simulink model "UAV_Hover_Sim"  (R2025b)
settings: Solver=VariableStepAuto  StartTime=0.0  StopTime=inf  RelTol=1e-3
undefined symbols (not defined in the file): A, b0, g, h, quad_m, rho_water, W, wc, wo
libraries: slpidlib x1, aerolibanimutils x1, uavutilslib x1
settings Model: Creator=Aorus PC  LastModifiedBy=David
settings OptimizationCC: ReuseModelBlockBuffer=off
settings DebuggingCC: UnderspecifiedInitializationDetection=Classic  MergeDetectMultiDrivingBlocksExec=none
settings ModelReferenceCC: PropagateSignalLabelsOutOfModel=off
settings RTWCC: GPUComputeCapability=3.5

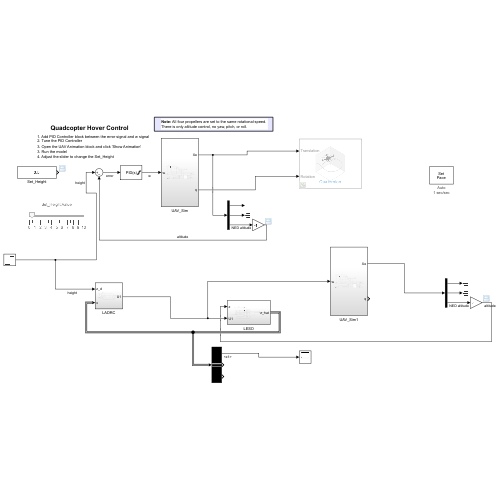
[thumbnail: Simulink's stored preview of the top-level diagram]
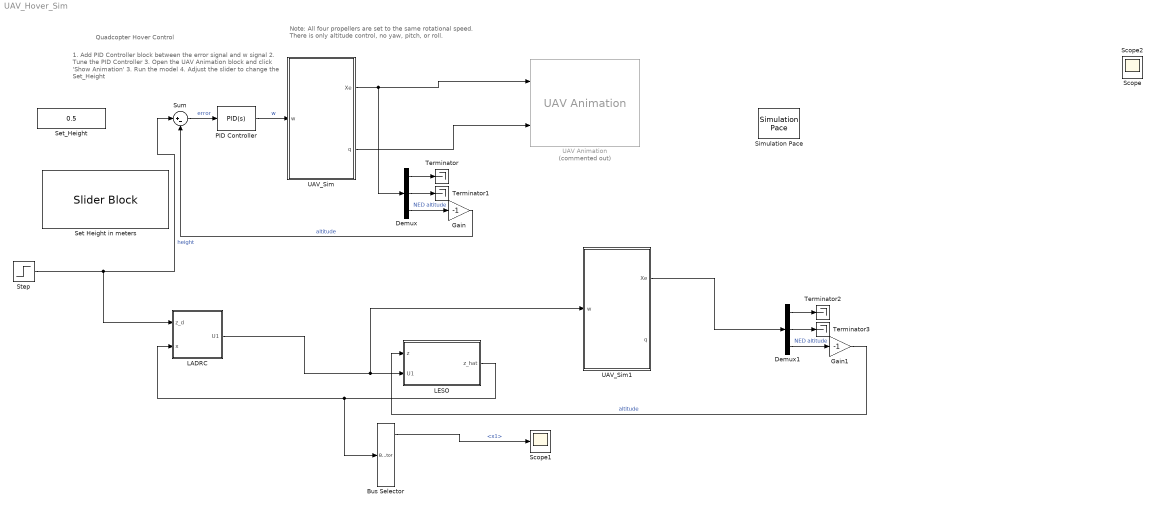
== system UAV_Hover_Sim ==
  note: Note: All four propellers are set to the same rotational speed.
      | There is only altitude control, no yaw, pitch, or roll.
  note: 1. Add PID Controller block between the error signal and w signal 2. Tune the PID Controller
      | 3. Open the UAV Animation block and click 'Show Animation'
      | 3. Run the model
      | 4. Adjust the slider to change the Set_Height
  note: Quadcopter Hover Control
  Bus Selector : BusSelector  OutputSignals=x1,x2,x3
  Demux : Demux  Outputs=3
  Demux1 : Demux  Outputs=3
  Gain : Gain  Gain=-1
  Gain1 : Gain  Gain=-1
  LADRC : Subsystem
  LESO : Subsystem
  PID Controller : slpidlib/PID Controller  Controller=PID  Form=Parallel  TimeDomain=Continuous-time  UseExternalTs=off  SampleTime=-1  IntegratorMethod=Forward Euler  FilterMethod=Forward Euler  ControllerParametersSource=internal  P=20  I=1  UseKiTs=off  D=40  UseExternalDerivativeSource=off  N=10  UseFilter=on  TunerSelectOption=Transfer Function Based (PID Tuner App)  InitialConditionSource=internal  InitialConditionForIntegrator=4000  InitialConditionForFilter=0  DifferentiatorICPrevScaledInput=0  ExternalReset=none  TrackingMode=off  Kt=1  LimitOutput=on  SatLimitsSource=internal  UpperSaturationLimit=10000  LowerSaturationLimit=0  LinearizeAsGain=on  AntiWindupMode=back-calculation  Kb=1  LimitIntegrator=on  UpperIntegratorSaturationLimit=10000  LowerIntegratorSaturationLimit=0  POutMin=[]  POutMax=[]  IOutMin=[]  IOutMax=[]  DOutMin=[]  DOutMax=[]  NOutMin=[]  NOutMax=[]  SumOutMin=[]  SumOutMax=[]  SaturationOutMin=[]  SaturationOutMax=[]  PParamMin=[]  PParamMax=[]  IParamMin=[]  IParamMax=[]  DParamMin=[]  DParamMax=[]  NParamMin=[]  NParamMax=[]  KbParamMin=[]  KbParamMax=[]  KtParamMin=[]  KtParamMax=[]  KbOutMin=[]  KbOutMax=[]  KtOutMin=[]  KtOutMax=[]  IntegratorOutMin=[]  IntegratorOutMax=[]  FilterOutMin=[]  FilterOutMax=[]  SumI1OutMin=[]  SumI1OutMax=[]  SumI2OutMin=[]  SumI2OutMax=[]  SumI3OutMin=[]  SumI3OutMax=[]  SumI4OutMin=[]  SumI4OutMax=[]  SumDOutMin=[]  SumDOutMax=[]  DifferentiatorOutMin=[]  DifferentiatorOutMax=[]  FilterDiffOutCoefMin=[]  FilterDiffOutCoefMax=[]  ReciprocalOutMin=[]  ReciprocalOutMax=[]  SumDenOutMin=[]  SumDenOutMax=[]  SumNumOutMin=[]  SumNumOutMax=[]  DivideOutMin=[]  DivideOutMax=[]  UdiffTsProdOutMin=[]  UdiffTsProdOutMax=[]  NTsProdOutMin=[]  NTsProdOutMax=[]  UintegralTsProdOutMin=[]  UintegralTsProdOutMax=[]  UngainTsProdOutMin=[]  UngainTsProdOutMax=[]  ClampingZeroOutDataTypeStr=Inherit: Inherit via back propagation  ClampingZeroOutMin=[]  ClampingZeroOutMax=[]  FilterDenConstantOutDataTypeStr=Inherit: Inherit via back propagation  FilterDenConstantOutMin=[]  FilterDenConstantOutMax=[]  PCopyOutDataTypeStr=Inherit: Inherit via back propagation  PCopyOutMin=[]  PCopyOutMax=[]  NCopyOutDataTypeStr=Inherit: Inherit via back propagation  NCopyOutMin=[]  NCopyOutMax=[]  IntegratorContinuousStateAttributes=''  IntegratorStateMustResolveToSignalObject=off  IntegratorRTWStateStorageClass=Auto  FilterContinuousStateAttributes=''  FilterStateMustResolveToSignalObject=off  FilterRTWStateStorageClass=Auto  ParallelPVariant=InternalParameters  IdealPVariant=Disabled  IVariant=InternalParameters  DVariant=InternalParameters  IntegratorVariant=Continuous  SatVariant=Enabled  AWVariant=BackCalculation  PCopyVariant=Disabled  TRVariant=Disabled  FdbkBlocksVariant=Forward  IdealPFdbkVariant=Disabled  SatFdbkVariant=Disabled  DerivativeFilterVariant=ContFilter  NVariant=InternalParameters  NCopyVariant=Disabled  FilterICVariant=InternalICsFilter  IntegratorICVariant=InternalICs  ExternalResetVariant=Disabled  TRSumVariant=Passthrough  SumFdbkVariant=Disabled  SumVariant=Sum_PID  TsampFilterVariant=InternalTs  TsampNgainVariant=Passthrough  TsampIntegralVariant=Disabled_SignalSpec  ExternalSaturationOutDataTypeStr=Inherit: Same as second input  DerivativeSourceVariant=ErrorSignal  PreIntVariant=InternalPreInt
  Scope1 : Scope
      settings: ActiveDisplayYMinimum=-1  ActiveDisplayYMaximum=1  DataLoggingVariableName=ScopeData3
  Set Height in meters : SliderBlock  ScaleMax=10  TickInterval=1
  Set_Height : Constant  Value=0.5
  Simulation Pace : aerolibanimutils/Simulation Pace  SimulationPace=1  SleepMode=Auto  OutputPaceError=off  SampleTime=1/30
  Step : Step  Time=10  Before=0.1  After=0.5  SampleTime=0
  Sum : Sum  Inputs=|+-
  Terminator{,1..3} (4 alike) : Terminator
  UAV Animation : uavutilslib/UAV Animation  Commented=on  NumUAV=1  DynamicUAVConfig=off  UAVType=Multirotor  UAVSize=4  UAVColor=[1 0 0]  UAVTrajectoryAlpha=1  InertialZDirection=Down  RotationFormat=Quaternion  DrawMarkers=off  SampleTime=-1
  UAV_Sim : Subsystem
  UAV_Sim1 : Subsystem
  Scope : Scope
      settings: TimeSpan=20  ActiveDisplayYMinimum=0.050000000000000017  ActiveDisplayYMaximum=0.55  YLabel=Altitude (m)
  Scope2 : Scope
      settings: ActiveDisplayYMinimum=0.03970156153398724  ActiveDisplayYMaximum=0.69900672000541475
  wires:
  UAV_Sim/1(Xe) -> Demux/1, UAV Animation/1
  UAV_Sim/2(q) -> UAV Animation/2
  Demux/1 -> Terminator/1
  Demux/2 -> Terminator1/1
  Gain/1 -> Sum/2  "altitude"
  Step/1 -> Sum/1, LADRC/1(z_d)  "height"
  Demux/3 -> Gain/1  "NED altitude"
  PID Controller/1 -> UAV_Sim/1(w)  "w"
  Sum/1 -> PID Controller/1  "error"
  LESO/1(z_hat) -> Bus Selector/1, LADRC/2(x)
  LADRC/1(U1) -> UAV_Sim1/1(w), LESO/2(U1)
  Demux1/3 -> Gain1/1  "NED altitude"
  Demux1/2 -> Terminator3/1
  Demux1/1 -> Terminator2/1
  UAV_Sim1/1(Xe) -> Demux1/1
  Gain1/1 -> LESO/1(z)  "altitude"
  Bus Selector/1 -> Scope1/1  "<x1>"

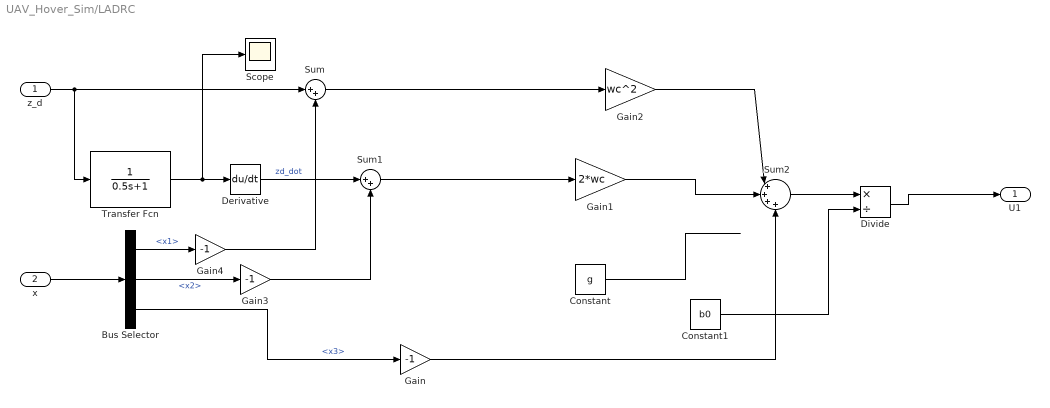
== system UAV_Hover_Sim/LADRC ==
  z_d : Inport
  x : Inport  Port=2
  Bus Selector : BusSelector  OutputSignals=x1,x2,x3
  Constant : Constant  Value=g
  Constant1 : Constant  Value=b0
  Derivative : Derivative
  Divide : Product  Inputs=*/
  Gain : Gain  Gain=-1
  Gain1 : Gain  Gain=2*wc
  Gain2 : Gain  Gain=wc^2
  Gain3 : Gain  Gain=-1
  Gain4 : Gain  Gain=-1
  Scope : Scope
      settings: ActiveDisplayYMinimum=-0.062471408438539523  ActiveDisplayYMaximum=0.56224267594685584  DataLoggingVariableName=ScopeData6
  Sum : Sum  Inputs=|++
  Sum1 : Sum  Inputs=|++
  Sum2 : Sum  Inputs=|++++
  Transfer Fcn : TransferFcn  Denominator=[0.5 1]
  U1 : Outport
  wires:
  Sum2/1 -> Divide/1
  x/1 -> Bus Selector/1
  Bus Selector/3 -> Gain/1  "<x3>"
  Gain2/1 -> Sum2/1
  Constant/1 -> ?
  Gain/1 -> Sum2/4
  Gain1/1 -> Sum2/2
  Bus Selector/1 -> Gain4/1  "<x1>"
  Bus Selector/2 -> Gain3/1  "<x2>"
  Transfer Fcn/1 -> Scope/1, Derivative/1
  z_d/1 -> Transfer Fcn/1, Sum/1
  Gain4/1 -> Sum/2
  Gain3/1 -> Sum1/2
  Derivative/1 -> Sum1/1  "zd_dot"
  Sum1/1 -> Gain1/1
  Sum/1 -> Gain2/1
  Divide/1 -> U1/1
  Constant1/1 -> Divide/2

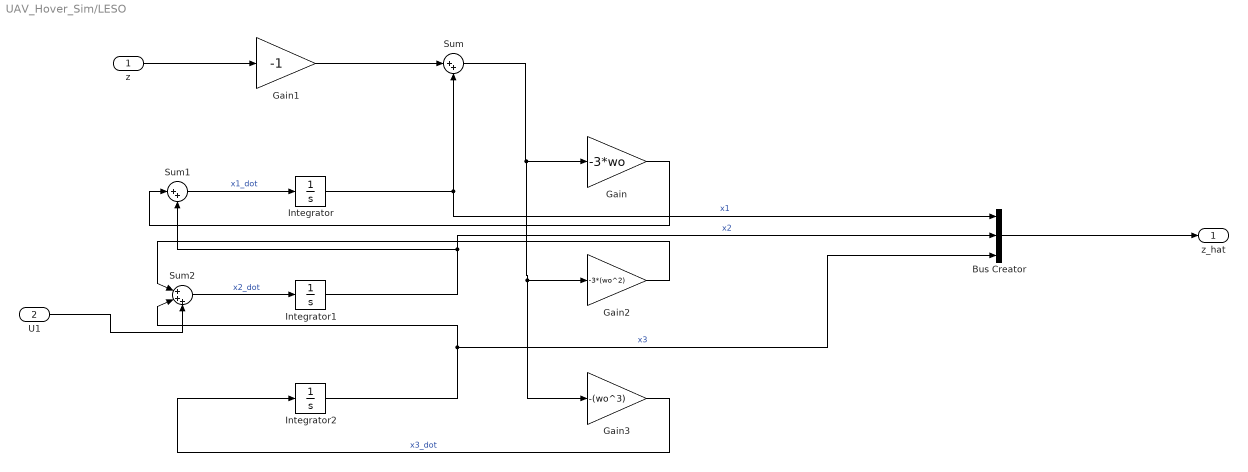
== system UAV_Hover_Sim/LESO ==
  z : Inport
  U1 : Inport  Port=2
  Bus Creator : BusCreator  Inputs=3
  Gain : Gain  Gain=-3*wo
  Gain1 : Gain  Gain=-1
  Gain2 : Gain  Gain=-3*(wo^2)
  Gain3 : Gain  Gain=-(wo^3)
  Integrator : Integrator  InitialCondition=0.1
  Integrator1 : Integrator
  Integrator2 : Integrator
  Sum : Sum  Inputs=|++
  Sum1 : Sum  Inputs=|++
  Sum2 : Sum  Inputs=|+++
  z_hat : Outport
  wires:
  z/1 -> Gain1/1
  Gain1/1 -> Sum/1
  Sum/1 -> Gain3/1, Gain2/1, Gain/1
  Integrator/1 -> Sum/2, Bus Creator/1  "x1"
  Gain3/1 -> Integrator2/1  "x3_dot"
  Bus Creator/1 -> z_hat/1
  Sum1/1 -> Integrator/1  "x1_dot"
  Gain/1 -> Sum1/1
  Integrator1/1 -> Bus Creator/2, Sum1/2  "x2"
  Integrator2/1 -> Bus Creator/3, Sum2/2  "x3"
  Gain2/1 -> Sum2/1
  Sum2/1 -> Integrator1/1  "x2_dot"
  U1/1 -> Sum2/3

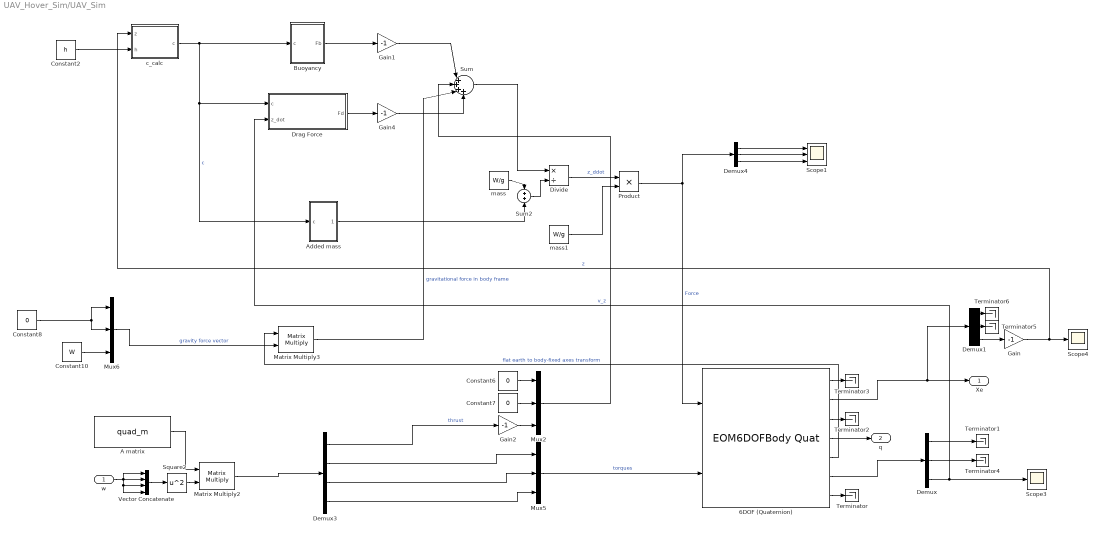
== system UAV_Hover_Sim/UAV_Sim ==
  w : Inport
  6DOF (Quaternion) : EOM6DOFBodyQuat  xme_0=[0 0 -0.1]
  A matrix : Constant  Value=quad_m
  Added mass : Subsystem
  Buoyancy : Subsystem
  Constant10 : Constant  Value=W
  Constant2 : Constant  Value=h
  Constant6 : Constant  Value=0
  Constant7 : Constant  Value=0
  Constant8 : Constant  Value=0
  Demux : Demux  Outputs=3
  Demux1 : Demux  Outputs=3
  Demux3 : Demux
  Demux4 : Demux  Outputs=3
  Divide : Product  Inputs=*/
  Drag Force : Subsystem
  Gain{,1..2,4} (4 alike) : Gain  Gain=-1
  Matrix Multiply2 : Product  Multiplication=Matrix(*)
  Matrix Multiply3 : Product  Multiplication=Matrix(*)
  Mux2 : Mux  Inputs=3
  Mux5 : Mux  Inputs=3
  Mux6 : Mux  Inputs=3
  Product : Product
  Scope1 : Scope  NumInputPorts=3
      settings: ActiveDisplayYMinimum=-36.152713090020676  ActiveDisplayYMaximum=4.0485705656672808  DataLoggingVariableName=ScopeData2
  Scope3 : Scope
      settings: ActiveDisplayYMinimum=-1  ActiveDisplayYMaximum=1  DataLoggingVariableName=ScopeData4
  Scope4 : Scope
      settings: ActiveDisplayYMinimum=-1  ActiveDisplayYMaximum=1  DataLoggingVariableName=ScopeData5
  Square2 : Math  Operator=square
  Sum : Sum  Inputs=|++++
  Sum2 : Sum
  Terminator{,1..6} (7 alike) : Terminator
  Vector Concatenate : Concatenate  NumInputs=4
  c_calc : MATLAB Function  TreatAsAtomicUnit=on
  mass : Constant  Value=W/g
  mass1 : Constant  Value=W/g
  Xe : Outport
  q : Outport  Port=2
  wires:
  Matrix Multiply3/1 -> Sum/3  "gravitational force in body frame"
  Demux4/1 -> Scope1/1
  Mux6/1 -> Matrix Multiply3/2  "gravity force vector"
  Constant10/1 -> Mux6/3
  Demux4/2 -> Scope1/2
  A matrix/1 -> Matrix Multiply2/1
  Demux3/1 -> Gain2/1  "thrust"
  Square2/1 -> Matrix Multiply2/2
  Matrix Multiply2/1 -> Demux3/1
  Demux3/2 -> Mux5/1
  Demux3/3 -> Mux5/2
  Demux3/4 -> Mux5/3
  Constant8/1 -> Mux6/1, Mux6/2
  Constant6/1 -> Mux2/1
  Constant7/1 -> Mux2/2
  Gain2/1 -> Mux2/3
  Demux4/3 -> Scope1/3
  w/1 -> Vector Concatenate/4, Vector Concatenate/3, Vector Concatenate/1, Vector Concatenate/2
  6DOF (Quaternion)/4 -> q/1
  6DOF (Quaternion)/5 -> Matrix Multiply3/1  "flat earth to body-fixed axes transform"
  6DOF (Quaternion)/2 -> Demux1/1, Xe/1
  Vector Concatenate/1 -> Square2/1
  Mux5/1 -> 6DOF (Quaternion)/2  "torques"
  6DOF (Quaternion)/7 -> Terminator/1
  6DOF (Quaternion)/6 -> Demux/1
  6DOF (Quaternion)/3 -> Terminator2/1
  6DOF (Quaternion)/1 -> Terminator3/1
  Constant2/1 -> c_calc/2(h)
  Product/1 -> 6DOF (Quaternion)/1, Demux4/1  "Force"
  mass/1 -> Sum2/1
  Drag Force/1(Fd) -> Gain4/1
  Buoyancy/1(Fb) -> Gain1/1
  Added mass/1(m_a) -> Sum2/2
  Sum/1 -> Divide/1
  Sum2/1 -> Divide/2
  c_calc/1(c) -> Drag Force/1(c), Added mass/1(c), Buoyancy/1(c)  "c"
  Demux/3 -> Drag Force/2(z_dot), Scope3/1  "v_z"
  Demux1/3 -> Gain/1
  Gain/1 -> c_calc/1(z), Scope4/1  "z"
  Demux/1 -> Terminator1/1
  Demux/2 -> Terminator4/1
  Demux1/2 -> Terminator5/1
  Demux1/1 -> Terminator6/1
  mass1/1 -> Product/2
  Divide/1 -> Product/1  "z_ddot"
  Mux2/1 -> Sum/2
  Gain4/1 -> Sum/4
  Gain1/1 -> Sum/1

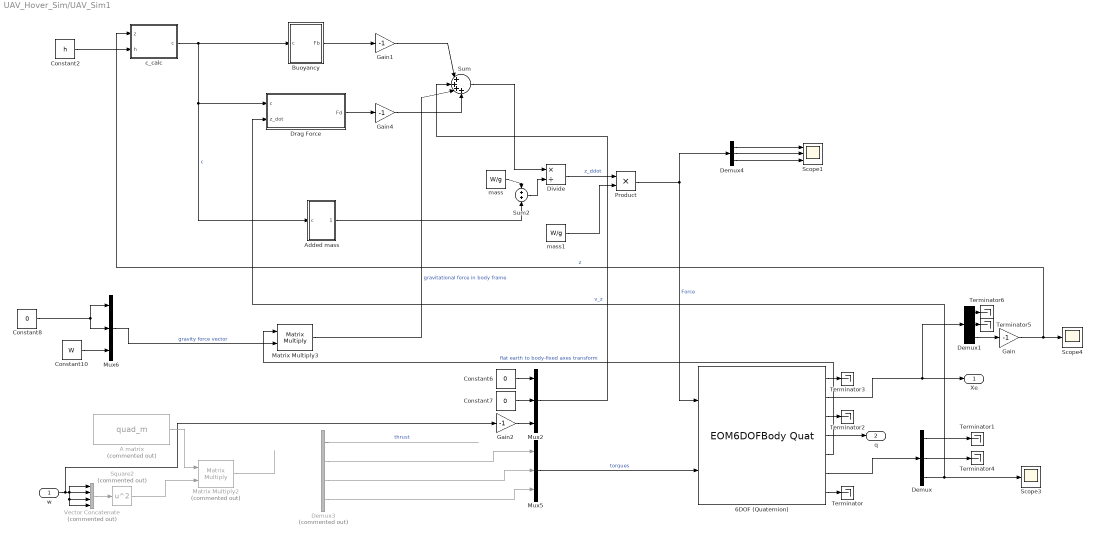
== system UAV_Hover_Sim/UAV_Sim1 ==
  w : Inport
  6DOF (Quaternion) : EOM6DOFBodyQuat  xme_0=[0 0 -0.1]
  A matrix : Constant  Commented=on  Value=quad_m
  Added mass : Subsystem
  Buoyancy : Subsystem
  Constant10 : Constant  Value=W
  Constant2 : Constant  Value=h
  Constant6 : Constant  Value=0
  Constant7 : Constant  Value=0
  Constant8 : Constant  Value=0
  Demux : Demux  Outputs=3
  Demux1 : Demux  Outputs=3
  Demux3 : Demux  Commented=on
  Demux4 : Demux  Outputs=3
  Divide : Product  Inputs=*/
  Drag Force : Subsystem
  Gain{,1..2,4} (4 alike) : Gain  Gain=-1
  Matrix Multiply2 : Product  Commented=on  Multiplication=Matrix(*)
  Matrix Multiply3 : Product  Multiplication=Matrix(*)
  Mux2 : Mux  Inputs=3
  Mux5 : Mux  Inputs=3
  Mux6 : Mux  Inputs=3
  Product : Product
  Scope1 : Scope  NumInputPorts=3
      settings: ActiveDisplayYMinimum=-36.152713090020676  ActiveDisplayYMaximum=4.0485705656672808  DataLoggingVariableName=ScopeData2
  Scope3 : Scope
      settings: ActiveDisplayYMinimum=-1  ActiveDisplayYMaximum=1  DataLoggingVariableName=ScopeData4
  Scope4 : Scope
      settings: ActiveDisplayYMinimum=-1  ActiveDisplayYMaximum=1  DataLoggingVariableName=ScopeData5
  Square2 : Math  Commented=on  Operator=square
  Sum : Sum  Inputs=|++++
  Sum2 : Sum
  Terminator{,1..6} (7 alike) : Terminator
  Vector Concatenate : Concatenate  Commented=on  NumInputs=4
  c_calc : MATLAB Function  TreatAsAtomicUnit=on
  mass : Constant  Value=W/g
  mass1 : Constant  Value=W/g
  Xe : Outport
  q : Outport  Port=2
  wires:
  Gain1/1 -> Sum/1
  Gain4/1 -> Sum/4
  Mux2/1 -> Sum/2
  Divide/1 -> Product/1  "z_ddot"
  mass1/1 -> Product/2
  Demux1/1 -> Terminator6/1
  Demux1/2 -> Terminator5/1
  Demux/2 -> Terminator4/1
  Demux/1 -> Terminator1/1
  Gain/1 -> Scope4/1, c_calc/1(z)  "z"
  Demux1/3 -> Gain/1
  Demux/3 -> Scope3/1, Drag Force/2(z_dot)  "v_z"
  c_calc/1(c) -> Buoyancy/1(c), Added mass/1(c), Drag Force/1(c)  "c"
  Sum2/1 -> Divide/2
  Sum/1 -> Divide/1
  Added mass/1(m_a) -> Sum2/2
  Buoyancy/1(Fb) -> Gain1/1
  Drag Force/1(Fd) -> Gain4/1
  mass/1 -> Sum2/1
  Product/1 -> Demux4/1, 6DOF (Quaternion)/1  "Force"
  Constant2/1 -> c_calc/2(h)
  6DOF (Quaternion)/1 -> Terminator3/1
  6DOF (Quaternion)/3 -> Terminator2/1
  6DOF (Quaternion)/6 -> Demux/1
  6DOF (Quaternion)/7 -> Terminator/1
  Mux5/1 -> 6DOF (Quaternion)/2  "torques"
  Vector Concatenate/1 -> Square2/1
  6DOF (Quaternion)/2 -> Xe/1, Demux1/1
  6DOF (Quaternion)/5 -> Matrix Multiply3/1  "flat earth to body-fixed axes transform"
  6DOF (Quaternion)/4 -> q/1
  w/1 -> Gain2/1, Vector Concatenate/2, Vector Concatenate/1, Vector Concatenate/3, Vector Concatenate/4
  Demux4/3 -> Scope1/3
  Gain2/1 -> Mux2/3
  Constant7/1 -> Mux2/2
  Constant6/1 -> Mux2/1
  Constant8/1 -> Mux6/2, Mux6/1
  Demux3/4 -> Mux5/3
  Demux3/3 -> Mux5/2
  Demux3/2 -> Mux5/1
  Matrix Multiply2/1 -> ?
  Square2/1 -> Matrix Multiply2/2
  Demux3/1 -> ?  "thrust"
  A matrix/1 -> Matrix Multiply2/1
  Demux4/2 -> Scope1/2
  Constant10/1 -> Mux6/3
  Mux6/1 -> Matrix Multiply3/2  "gravity force vector"
  Demux4/1 -> Scope1/1
  Matrix Multiply3/1 -> Sum/3  "gravitational force in body frame"

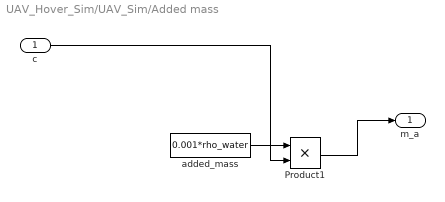
== system UAV_Hover_Sim/UAV_Sim/Added mass ==
  c : Inport
  Product1 : Product
  added_mass : Constant  Value=0.001*rho_water
  m_a : Outport
  wires:
  c/1 -> Product1/2
  Product1/1 -> m_a/1
  added_mass/1 -> Product1/1

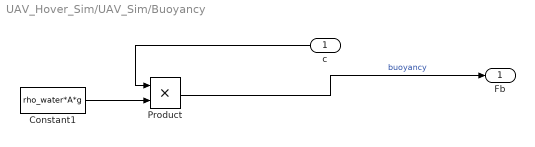
== system UAV_Hover_Sim/UAV_Sim/Buoyancy ==
  c : Inport
  Constant1 : Constant  Value=rho_water*A*g
  Product : Product
  Fb : Outport
  wires:
  Product/1 -> Fb/1  "buoyancy"
  c/1 -> Product/1
  Constant1/1 -> Product/2

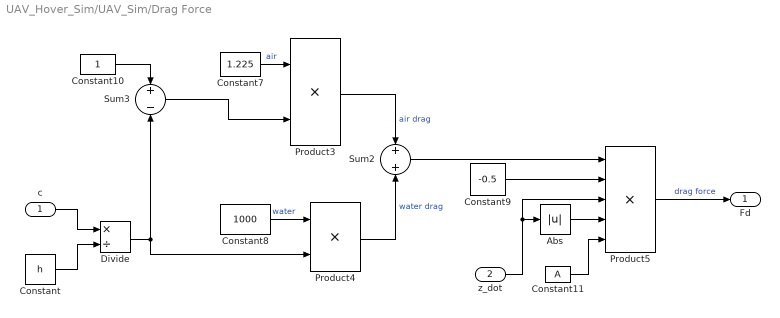
== system UAV_Hover_Sim/UAV_Sim/Drag Force ==
  c : Inport
  z_dot : Inport  Port=2
  Abs : Abs  SaturateOnIntegerOverflow=off
  Constant : Constant  Value=h
  Constant10 : Constant
  Constant11 : Constant  Value=A
  Constant7 : Constant  Value=1.225
  Constant8 : Constant  Value=1000
  Constant9 : Constant  Value=-0.5
  Divide : Product  Inputs=*/
  Product3 : Product
  Product4 : Product
  Product5 : Product  Inputs=5
  Sum2 : Sum
  Sum3 : Sum  Inputs=+-
  Fd : Outport
  wires:
  Constant/1 -> Divide/2
  c/1 -> Divide/1
  Constant7/1 -> Product3/1  "air"
  Product3/1 -> Sum2/1  "air drag"
  Abs/1 -> Product5/4
  z_dot/1 -> Product5/3, Abs/1
  Constant9/1 -> Product5/2
  Sum2/1 -> Product5/1
  Constant10/1 -> Sum3/1
  Constant8/1 -> Product4/1  "water"
  Sum3/1 -> Product3/2
  Constant11/1 -> Product5/5
  Product4/1 -> Sum2/2  "water drag"
  Product5/1 -> Fd/1  "drag force"
  Divide/1 -> Product4/2, Sum3/2

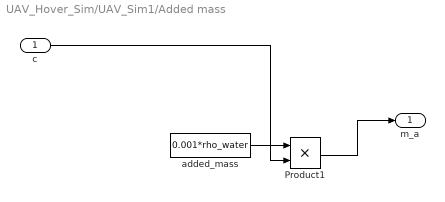
== system UAV_Hover_Sim/UAV_Sim1/Added mass ==
  c : Inport
  Product1 : Product
  added_mass : Constant  Value=0.001*rho_water
  m_a : Outport
  wires:
  added_mass/1 -> Product1/1
  Product1/1 -> m_a/1
  c/1 -> Product1/2

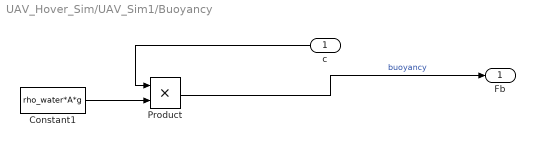
== system UAV_Hover_Sim/UAV_Sim1/Buoyancy ==
  c : Inport
  Constant1 : Constant  Value=rho_water*A*g
  Product : Product
  Fb : Outport
  wires:
  Constant1/1 -> Product/2
  c/1 -> Product/1
  Product/1 -> Fb/1  "buoyancy"

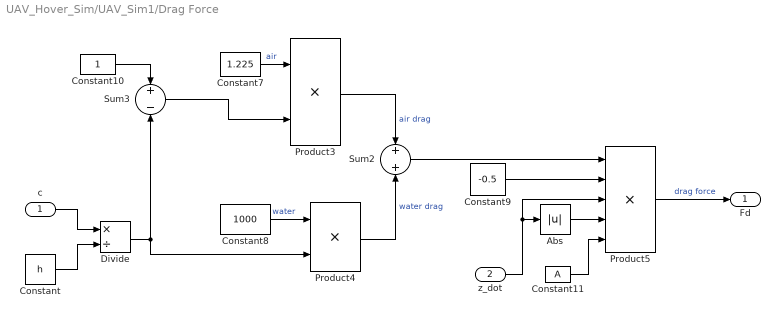
== system UAV_Hover_Sim/UAV_Sim1/Drag Force ==
  c : Inport
  z_dot : Inport  Port=2
  Abs : Abs  SaturateOnIntegerOverflow=off
  Constant : Constant  Value=h
  Constant10 : Constant
  Constant11 : Constant  Value=A
  Constant7 : Constant  Value=1.225
  Constant8 : Constant  Value=1000
  Constant9 : Constant  Value=-0.5
  Divide : Product  Inputs=*/
  Product3 : Product
  Product4 : Product
  Product5 : Product  Inputs=5
  Sum2 : Sum
  Sum3 : Sum  Inputs=+-
  Fd : Outport
  wires:
  Divide/1 -> Sum3/2, Product4/2
  Product5/1 -> Fd/1  "drag force"
  Product4/1 -> Sum2/2  "water drag"
  Constant11/1 -> Product5/5
  Sum3/1 -> Product3/2
  Constant8/1 -> Product4/1  "water"
  Constant10/1 -> Sum3/1
  Sum2/1 -> Product5/1
  Constant9/1 -> Product5/2
  z_dot/1 -> Abs/1, Product5/3
  Abs/1 -> Product5/4
  Product3/1 -> Sum2/1  "air drag"
  Constant7/1 -> Product3/1  "air"
  c/1 -> Divide/1
  Constant/1 -> Divide/2

== matlab function UAV_Hover_Sim/UAV_Sim/c_calc ==
  data: z input; c output; h input
function c = fcn(z, h)

if z > h/2
    c = 0;
elseif z < -h/2
    c = h;
else 
    c = h/2 - z;
end

== matlab function UAV_Hover_Sim/UAV_Sim1/c_calc ==
  data: z input; c output; h input
function c = fcn(z, h)

if z > h/2
    c = 0;
elseif z < -h/2
    c = h;
else 
    c = h/2 - z;
end
